simulink model "R1_boiler_model"  (R2025a)
settings: Solver=VariableStepAuto  StartTime=0.0  StopTime=0  RelTol=1e-3
settings Model: Creator=Krithik  LastModifiedBy=Krithik

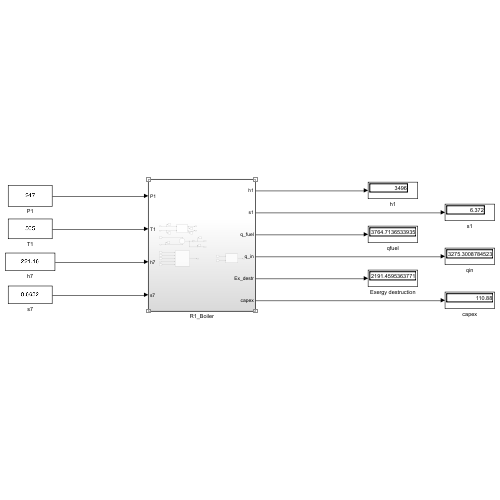
[thumbnail: Simulink's stored preview of the top-level diagram]
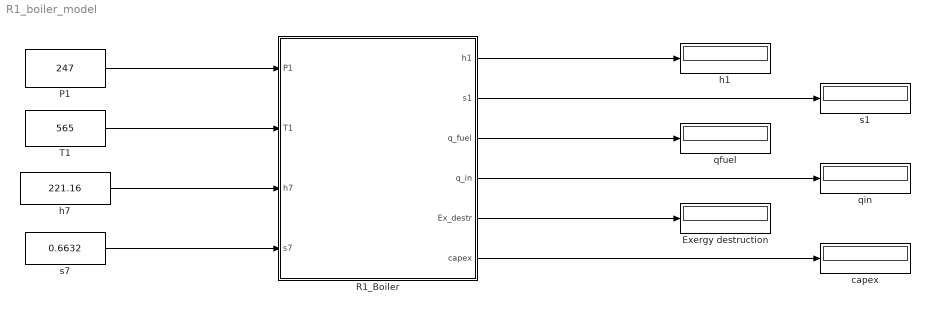
== system R1_boiler_model ==
  Exergy destruction : Display
  P1 : Constant  Value=247
  R1_Boiler : Subsystem
  T1 : Constant  Value=565
  capex : Display
  h1 : Display
  h7 : Constant  Value=221.16
  qfuel : Display
  qin : Display
  s1 : Display
  s7 : Constant  Value=0.6632
  wires:
  P1/1 -> R1_Boiler/1(P1)
  T1/1 -> R1_Boiler/2(T1)
  h7/1 -> R1_Boiler/3(h7)
  s7/1 -> R1_Boiler/4(s7)
  R1_Boiler/1(h1) -> h1/1
  R1_Boiler/2(s1) -> s1/1
  R1_Boiler/3(q_fuel) -> qfuel/1
  R1_Boiler/4(q_in) -> qin/1
  R1_Boiler/5(Ex_destr) -> Exergy destruction/1
  R1_Boiler/6(capex) -> capex/1

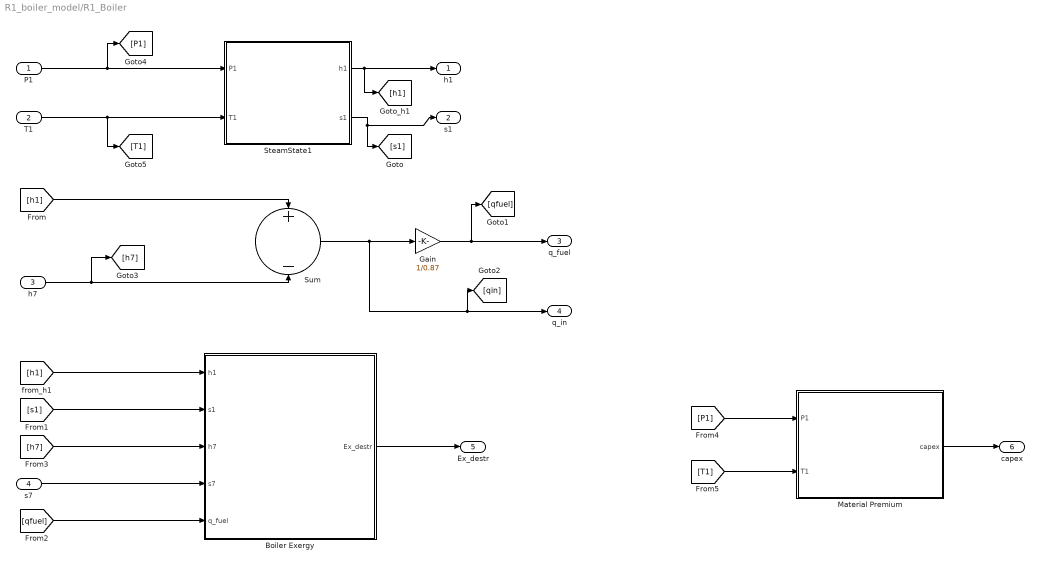
== system R1_boiler_model/R1_Boiler ==
  P1 : Inport
  T1 : Inport  Port=2
  h7 : Inport  Port=3
  s7 : Inport  Port=4
  Boiler Exergy : MATLAB Function  TreatAsAtomicUnit=on
  Gain : Gain  Gain=1/0.87
  Material Premium : MATLAB Function  TreatAsAtomicUnit=on
  SteamState1 : MATLAB Function  TreatAsAtomicUnit=on
  Sum : Sum  Inputs=+-
  h1 : Outport
  s1 : Outport  Port=2
  q_fuel : Outport  Port=3
  q_in : Outport  Port=4
  Ex_destr : Outport  Port=5
  capex : Outport  Port=6
  wires:
  SteamState1/2(s1) -> s1/1, [s1]
  T1/1 -> [T1], SteamState1/2(T1)
  [T1] -> Material Premium/2(T1)
  Sum/1 -> q_in/1, [qin], Gain/1
  [h7] -> Boiler Exergy/3(h7)
  SteamState1/1(h1) -> h1/1, [h1]
  Gain/1 -> q_fuel/1, [qfuel]
  [s1] -> Boiler Exergy/2(s1)
  h7/1 -> [h7], Sum/2
  [h1] -> Sum/1
  [P1] -> Material Premium/1(P1)
  [h1] -> Boiler Exergy/1(h1)
  P1/1 -> [P1], SteamState1/1(P1)
  [qfuel] -> Boiler Exergy/5(q_fuel)
  Boiler Exergy/1(Ex_destr) -> Ex_destr/1
  s7/1 -> Boiler Exergy/4(s7)
  Material Premium/1(capex) -> capex/1

== matlab function R1_boiler_model/R1_Boiler/Boiler Exergy ==
  data: h1 input; Ex_destr output; s1 input; h7 input; s7 input; q_fuel input
function Ex_destr = fcn(h1, s1, h7, s7, q_fuel)
coder.extrinsic('props_pT_for_simulink');
h0 = 0; s0 = 0;
[h0, s0] = props_pT_for_simulink(1.013, 25);
T0 = 298.15; phi = 1.0;
psi1 = (h1 - h0) - T0*(s1 - s0);
psi7 = (h7 - h0) - T0*(s7 - s0);
Ex_destr = phi*q_fuel - (psi1 - psi7);

== matlab function R1_boiler_model/R1_Boiler/SteamState1 ==
  data: P1 input; h1 output; T1 input; s1 output
function [h1, s1] = fcn(P1, T1)
coder.extrinsic('props_pT_for_simulink');
h1 = 0; s1 = 0;
[h1, s1] = props_pT_for_simulink(P1, T1);

== matlab function R1_boiler_model/R1_Boiler/Material Premium ==
  data: P1 input; capex output; T1 input
function capex = fcn(P1, T1)
boiler_share = 0.35;  capex_base = 8*660;
if T1 <= 566
    tprem = 0;
elseif T1 <= 600
    tprem = 0.06;
elseif T1 <= 620
    tprem = 0.15;
else
    tprem = 0.30;
end
pprem = 5e-4*max(P1 - 247, 0);
capex = boiler_share*capex_base*(tprem + pprem);
